simulink model "HW4"  (R2022b)
settings: Solver=FixedStepAuto  StartTime=0.0  StopTime=1500  FixedStep=0.001  RelTol=1e-3
libraries: simulink x1
settings Model: Creator=ali14  LastModifiedBy=ali14

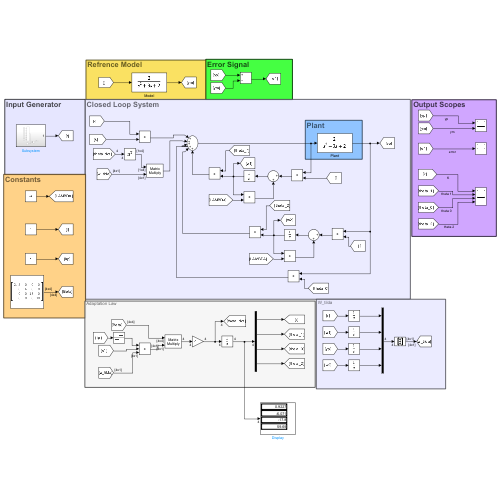
[thumbnail: Simulink's stored preview of the top-level diagram]
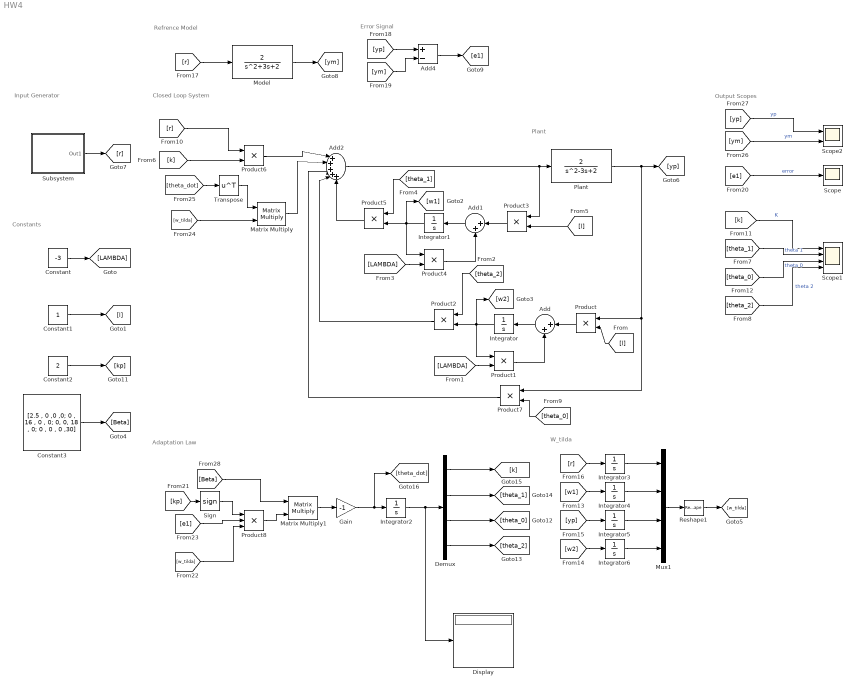
== system HW4 ==
  note: Constants
  note: W_tilda
  note: Adaptation Law
  note: Closed Loop System
  note: Plant
  note: Refrence Model
  note: Error Signal
  note: Input Generator
  note: Output Scopes
  Add : Sum  Inputs=|++
  Add1 : Sum  Inputs=|++
  Add2 : Sum  Inputs=|+++++
  Add4 : Sum  Inputs=+-
  Constant : Constant  Value=-3
  Constant1 : Constant
  Constant2 : Constant  Value=2
  Constant3 : Constant  Value=[2.5 , 0 ,0 ,0; 0 , 16 , 0 , 0; 0, 0, 18 , 0; 0 , 0 , 0 ,30]
  Demux : Demux
  Display : Display
  Gain : Gain  Gain=-1
  Integrator{,1..6} (7 alike) : Integrator
  Matrix Multiply : Product  Multiplication=Matrix(*)
  Matrix Multiply1 : Product  Multiplication=Matrix(*)
  Model : TransferFcn  Numerator=[2]  Denominator=[1 3 2]
  Mux1 : Mux
  Plant : TransferFcn  Numerator=[2]  Denominator=[1 -3 2]
  Product{,1..7} (8 alike) : Product
  Product8 : Product  Inputs=3
  Reshape1 : Reshape  OutputDimensionality=Column vector (2-D)
  Scope : Scope
  Scope1 : Scope  NumInputPorts=4
  Scope2 : Scope  NumInputPorts=2
  Sign : Signum
  Subsystem : Subsystem
  Transpose : Math  Operator=transpose
  wires:
  [yp] -> Scope2/1  "yp"
  [ym] -> Scope2/2  "ym"
  [e1] -> Scope/1  "error"
  [k] -> Scope1/1  "K"
  Integrator6/1 -> Mux1/4
  Integrator5/1 -> Mux1/3
  Integrator4/1 -> Mux1/2
  Integrator3/1 -> Mux1/1
  Matrix Multiply/1 -> Add2/2
  Transpose/1 -> Matrix Multiply/1
  [w_tilda] -> Matrix Multiply/2
  [theta_dot] -> Transpose/1
  [k] -> Product6/2
  [r] -> Product6/1
  Plant/1 -> [yp], Product7/1, Product/1
  Product6/1 -> Add2/1
  Product2/1 -> Add2/4
  Product3/1 -> Add1/1
  Mux1/1 -> Reshape1/1
  Sign/1 -> Product8/1
  Product4/1 -> Add1/2
  Demux/1 -> [k]
  Add2/1 -> Product3/1, Plant/1
  [theta_0] -> Product7/2
  [e1] -> Product8/2
  Demux/2 -> [theta_1]
  [yp] -> Integrator5/1
  [LAMBDA] -> Product4/2
  [w2] -> Integrator6/1
  [yp] -> Add4/1
  Constant2/1 -> [kp]
  Integrator2/1 -> Display/1, Demux/1
  [ym] -> Add4/2
  Model/1 -> [ym]
  Demux/4 -> [theta_2]
  Add/1 -> Integrator/1
  Demux/3 -> [theta_0]
  Product7/1 -> Add2/3
  Reshape1/1 -> [w_tilda]
  [theta_2] -> Scope1/4  "theta 2"
  Gain/1 -> [theta_dot], Integrator2/1
  [r] -> Model/1
  Product1/1 -> Add/2
  Add4/1 -> [e1]
  Product5/1 -> Add2/5
  [theta_0] -> Scope1/3  "theta 0"
  [theta_2] -> Product2/1
  [r] -> Integrator3/1
  [theta_1] -> Scope1/2  "theta 1"
  Constant/1 -> [LAMBDA]
  Integrator/1 -> [w2], Product2/2, Product1/1
  Integrator1/1 -> [w1], Product5/2, Product4/1
  Product/1 -> Add/1
  Add1/1 -> Integrator1/1
  [l] -> Product3/2
  Constant1/1 -> [l]
  [theta_1] -> Product5/1
  [l] -> Product/2
  [w1] -> Integrator4/1
  [kp] -> Sign/1
  [LAMBDA] -> Product1/2
  Constant3/1 -> [Beta]
  [w_tilda] -> Product8/3
  Product8/1 -> Matrix Multiply1/2
  Matrix Multiply1/1 -> Gain/1
  [Beta] -> Matrix Multiply1/1
  Subsystem/1(Out1) -> [r]

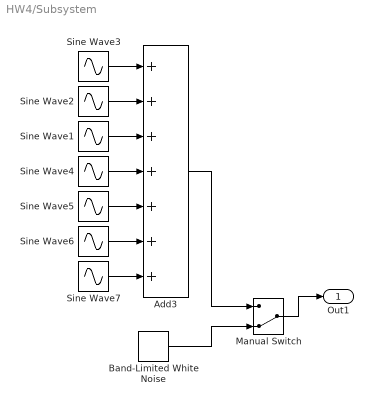
== system HW4/Subsystem ==
  Add3 : Sum  Inputs=+++++++
  Band-Limited White Noise : simulink/Sources/Band-Limited White Noise  Cov=[0.1]  Ts=0.1  seed=[23341]
  Manual Switch : ManualSwitch  CurrentSetting=0
  Sine Wave1 : Sin  Amplitude=3  Frequency=2  SampleTime=0
  Sine Wave2 : Sin  Amplitude=3  Frequency=1.5  SampleTime=0
  Sine Wave3 : Sin  Frequency=0.5  SampleTime=0
  Sine Wave4 : Sin  Amplitude=3  Frequency=3  SampleTime=0
  Sine Wave5 : Sin  Amplitude=3  Frequency=5  SampleTime=0
  Sine Wave6 : Sin  Amplitude=3  Frequency=1.5  SampleTime=0
  Sine Wave7 : Sin  Amplitude=3  Frequency=7  SampleTime=0
  Out1 : Outport
  wires:
  Sine Wave3/1 -> Add3/1
  Sine Wave2/1 -> Add3/2
  Add3/1 -> Manual Switch/1
  Manual Switch/1 -> Out1/1
  Band-Limited White Noise/1 -> Manual Switch/2
  Sine Wave5/1 -> Add3/5
  Sine Wave6/1 -> Add3/6
  Sine Wave7/1 -> Add3/7
  Sine Wave4/1 -> Add3/4
  Sine Wave1/1 -> Add3/3
